simulink model "ACFT11_a_121_flatearth_backup"  (R2026a)
settings: Solver=ode15s  StopTime=10  FixedStep=0.01  MaxStep=0.05  MinStep=1e-4  AbsTol=1e-4
model workspace (MAT data in the model file):
  op11 : opcond.OperatingPoint (value not decoded)
  op_trim1 : opcond.OperatingReport (value not decoded)
  op_trim12 : opcond.OperatingReport (value not decoded)
  op_trim15 : opcond.OperatingReport (value not decoded)
  op_trim16 : opcond.OperatingReport (value not decoded)
  op_trim17 : opcond.OperatingReport (value not decoded)
  op_trim18 : opcond.OperatingReport (value not decoded)
  op_trim2 : opcond.OperatingReport (value not decoded)
  op_trim20 : opcond.OperatingReport (value not decoded)
  op_trim21 : opcond.OperatingReport (value not decoded)
  op_trim22 : opcond.OperatingReport (value not decoded)
  op_trim23 : opcond.OperatingReport (value not decoded)
  op_trim24 : opcond.OperatingReport (value not decoded)
  op_trim25 : opcond.OperatingReport (value not decoded)
  op_trim29 : opcond.OperatingReport (value not decoded)
  op_trim3 : opcond.OperatingReport (value not decoded)
  op_trim30 : opcond.OperatingReport (value not decoded)
  op_trim4 : opcond.OperatingReport (value not decoded)
  op_trim40 : opcond.OperatingReport (value not decoded)
  op_trim42 : opcond.OperatingReport (value not decoded)
  op_trim5 : opcond.OperatingReport (value not decoded)
  op_trim50 : opcond.OperatingReport (value not decoded)
  op_trim7 : opcond.OperatingReport (value not decoded)
  op_trim9 : opcond.OperatingReport (value not decoded)
values from neighbouring files (symbols this model uses):
  b = min(1, 2*(1-frac))    [export_kml.m]    (also in flight_hud.m = chaseBack; inertiatensor62.m = 9.05; setup_bfl_analysis.m = 9.05; setup_fcs_sim.m = 9.05)
  c = bar_colors{min(k,numel(bar_colors))}    [analyze_bfl.m]    (also in ecef_eom_fcn.m = w_eb_b(3); inertiatensor62.m = 15.55; optimize_indi_gains.m = 15.55; restore_normal_fcs.m = 15.55)
  CL_AlphaDot = 0    [inertiatensor62.m]    (also in setup_bfl_analysis.m; setup_fcs_sim.m; setup_takeoff_fcs.m)
  Cm_AlphaDot = 0    [inertiatensor62.m]    (also in setup_bfl_analysis.m; setup_fcs_sim.m; setup_takeoff_fcs.m)
  F = convhull(pts)    [Visualization_Takeoff2.m]    (also in attitude_ribbon.m = {[1 2 3],[1 4 2],[1 4 3],[4 5 1]})
  FCS_aerospike_thrust = 250000.0    (= 250000)    [fcs_params.m]
  FCS_alpha_max = 16.0    (= 16)    [fcs_params.m]
  FCS_bank_max = 35.0    (= 35)    [fcs_params.m]
  FCS_da_max = 20.0    (= 20)    [fcs_params.m]
  FCS_de_max = 25.0    (= 25)    [fcs_params.m]
  FCS_dr_max = 25.0    (= 25)    [fcs_params.m]
  FCS_dt = 0.01    [fcs_params.m]
  FCS_g = 9.80665    [fcs_params.m]
  FCS_Gmin_p = 0.02    [fcs_params.m]
  FCS_Gmin_q = 0.02    [fcs_params.m]
  FCS_Gmin_r = 0.01    [fcs_params.m]
  FCS_h_gnd = 2.24    [fcs_params.m]
  FCS_hdot_max = 30.0    (= 30)    [fcs_params.m]
  FCS_hdot_td = 0.3    [fcs_params.m]
  FCS_Kalpha = 3.0    (= 3)    [fcs_params.m]
  FCS_Kalpha_lim = 2.0    (= 2)    [fcs_params.m]
  FCS_Kbeta = 2.0    (= 2)    [fcs_params.m]
  FCS_Kflare = 1.0    (= 1)    [fcs_params.m]
  FCS_Kgamma = 1.5    [fcs_params.m]
  FCS_Kh = 0.10    (= 0.1)    [fcs_params.m]
  FCS_Knz = 20.0    (= 20)    [fcs_params.m]
  FCS_Kp = 6.0    (= 6)    [fcs_params.m]
  FCS_Kphi = 3.0    (= 3)    [fcs_params.m]
  FCS_Kq = 5.0    (= 5)    [fcs_params.m]
  FCS_Kr = 4.0    (= 4)    [fcs_params.m]
  FCS_Ktheta = 2.0    (= 2)    [fcs_params.m]
  FCS_link_timeout = 1.0    (= 1)    [fcs_params.m]
  FCS_MODE_AUTO = 0    [fcs_params.m]
  FCS_Nfilt = 20.0    (= 20)    [fcs_params.m]
  FCS_Nz_max = 3.0    (= 3)    [fcs_params.m]
  FCS_Nz_min = -1.0    (= -1)    [fcs_params.m]
  FCS_p_max = 40.0    (= 40)    [fcs_params.m]
  FCS_q_max = 15.0    (= 15)    [fcs_params.m]
  FCS_qbar_hi = 6000.0    (= 6000)    [fcs_params.m]
  FCS_qbar_lo = 1000.0    (= 1000)    [fcs_params.m]
  FCS_r_max = 15.0    (= 15)    [fcs_params.m]
  FCS_relight_M_hi = 2.0    (= 2)    [fcs_params.m]
  FCS_relight_M_lo = 0.35    [fcs_params.m]
  FCS_relight_qbar = 3000.0    (= 3000)    [fcs_params.m]
  FCS_stick_detent = 0.03    [fcs_params.m]
  FCS_stick_p_scale = 60.0    (= 60)    [fcs_params.m]
  FCS_stick_q_scale = 15.0    (= 15)    [fcs_params.m]
  FCS_tau_flare = 3.0    (= 3)    [fcs_params.m]
  FCS_TECS_Kep = 0.25    [fcs_params.m]
  FCS_TECS_Ktp = 0.30    (= 0.3)    [fcs_params.m]
  FCS_theta_climb = 12.0    (= 12)    [fcs_params.m]
  FCS_theta_max = 30.0    (= 30)    [fcs_params.m]
  FCS_theta_min = -20.0    (= -20)    [fcs_params.m]
  FCS_theta_trim = 0.0    (= 0)    [fcs_params.m]
  FCS_thr_max = 1.0    (= 1)    [fcs_params.m]
  FCS_thr_min = 0.0    (= 0)    [fcs_params.m]
  FCS_thr_trim = 0.50    (= 0.5)    [fcs_params.m]
  FCS_V_rotate = 94.0    (= 94)    [fcs_params.m]
  FCS_Vmin = 60.0    (= 60)    [fcs_params.m]
  FF_rates = [0.0,              2.5,              5.0,             73.0,             78.0,              0.5]    [fcs_params.m]
  g = @(n,d) i_basevar(n,d)    [analyze_control_authority.m]    (also in export_kml.m = 1 - abs(2*frac-1); inertiatensor62.m = 9.80665; setup_bfl_analysis.m = 9.80665; setup_fcs_sim.m = 9.80665)
  GS_Gp_tab = Cl_da * (S*b/Ixx)    [setup_gschedule.m]
  GS_Gq_tab = Cm_de * (S*c/Iyy)    [setup_gschedule.m]
  GS_Gr_tab = Cn_dr * (S*b/Izz)    [setup_gschedule.m]
  MASS_fuel_total = MASS_full - MASS_empty - MASS_orbiter    (= 14700)    [fcs_params.m]
  q = q/norm(q)    [build_ecef_x0.m]    (also in ecef_eom_fcn.m = state(7:10); ecef_out_fcn.m = state(7:10); setup_ecef.m; test_ecef_eom.m = state(7:10))
  r = [0;diff(xc)]/0.1    [analyze_control_authority.m]    (also in ecef_eom_fcn.m = sqrt(r_e(1)^2+r_e(2)^2+r_e(3)^2); ecef_weight_body.m = sqrt(x^2 + y^2 + z^2); export_kml.m = min(1, 2*frac); test_ecef_eom.m = sqrt(r_e(1)^2+r_e(2)^2+r_e(3)^2))
  S = {'\delta_e',DE,lim.de,'b'; '\delta_a',DA,lim.da,[0 .6 0]; '\delta_r',DR,lim.dr,[.85 .3 .1]}    [analyze_control_authority.m]    (also in attitude_ribbon.m = load(char(src)); build_ecef_x0.m = sqrt(1+C(3,3)-C(1,1)-C(2,2))*2; export_kml.m = load(char(src)); flight_hud.m = load(char(src)))
  s = A.surfaces(i)    [analyze_control_authority.m]    (also in setup_propulsion.m = [s, sprintf(')
  y_cg = 0    [inertiatensor62.m]    (also in setup_bfl_analysis.m; setup_fcs_sim.m; setup_takeoff_fcs.m)
  z_cg = 0.0    (= 0)    [inertiatensor62.m]    (also in setup_bfl_analysis.m; setup_fcs_sim.m; setup_takeoff_fcs.m)
undefined symbols (not defined in the file or in its folder): deg, DiscIntNeverNeededParam, EqM, GS_alpha_cl, GS_alpha_cm, GS_alpha_cn, GS_mach_cl, GS_mach_cm, GS_mach_cn, MIL, Moderate, rad
libraries: aerolibconvert2 x21, simulink x7, aerolibfltsims x3, aerolibwind2 x3, aerolibanim x1, aerolibatmos2 x1, shareddyn x1, aerolibobsolete x1
(part 2 of 4)

== system ACFT11_a_121_flatearth_backup/WindModels ==
  h : Inport
  V : Inport  Port=2
  DCM : Inport  Port=3
  qbar : Inport  Port=4
  phase : Inport  Port=5
  DiscreteGust : aerolibwind2/Discrete Wind Gust Model  units=Metric (MKS)  Gx=on  Gy=on  Gz=on  t_0=WIND_gust_t0  d_m=WIND_gust_len  v_m=WIND_gust_amp
  Dryden Wind Turbulence Model (Discrete (+q +r)) : aerolibwind2/Dryden Wind Turbulence Model  (Continuous (+q -r))  units=Metric (MKS)  spec=MIL-F-8785C  model=Discrete Dryden (+q +r)  W20=WIND_W20  Wdeg=WIND_Wdeg  TurbProb=10^-3 - Moderate  L_high=WIND_Lhigh  Wingspan=FCS_b  ts=0.02  Seed=[23341 23342 23343 23344]  T_on=on
      settings: LibrarySourceBlock=|
      | aerolibwind2/Dryden Wind Turbulence Model
      | (Discrete (+q +r))
  MeanToBody : Product  Multiplication=Matrix(*)
  MeanWind : MATLAB Function  TreatAsAtomicUnit=on
  Scheduler : MATLAB Function  TreatAsAtomicUnit=on
  Vclamp : Saturate  UpperLimit=inf  LowerLimit=1
  WindShear : aerolibwind2/Wind Shear Model  units=Metric (MKS)  phase=Category C - Terminal Flight Phase  W_20=WIND_W20  Wdeg=WIND_Wdeg
  gDemux : Demux  Outputs=3
  pGust : Product
  pRate : Product
  pShear : Product
  pTurb : Product
  sWind : Sum  Inputs=++++
  WindBody : Outport
  GustRates : Outport  Port=2
  wires:
  V/1 -> Vclamp/1
  h/1 -> Dryden Wind Turbulence Model (Discrete (+q +r))/1, WindShear/1, MeanWind/1(h), Scheduler/3(h)
  Vclamp/1 -> Dryden Wind Turbulence Model (Discrete (+q +r))/2, DiscreteGust/1
  DCM/1 -> Dryden Wind Turbulence Model (Discrete (+q +r))/3, WindShear/2, MeanToBody/1
  MeanWind/1(W_ned) -> MeanToBody/2
  qbar/1 -> Scheduler/1(qbar)
  phase/1 -> Scheduler/2(phase)
  Scheduler/1(g) -> gDemux/1
  gDemux/1 -> pTurb/2, pRate/2
  gDemux/2 -> pGust/2
  gDemux/3 -> pShear/2
  Dryden Wind Turbulence Model (Discrete (+q +r))/1 -> pTurb/1
  Dryden Wind Turbulence Model (Discrete (+q +r))/2 -> pRate/1
  WindShear/1 -> pShear/1
  DiscreteGust/1 -> pGust/1
  MeanToBody/1 -> sWind/1
  pTurb/1 -> sWind/2
  pShear/1 -> sWind/3
  pGust/1 -> sWind/4
  sWind/1 -> WindBody/1
  pRate/1 -> GustRates/1

== system ACFT11_a_121_flatearth_backup/aerospike ==
  Manual Switch1 : ManualSwitch
  Scope1 : Scope
      settings: ActiveDisplayYMinimum=711.4  ActiveDisplayYMaximum=2711.4  DataLoggingVariableName=ScopeData8
  TotalWeight full : Constant  Value=24000
  TotalWeightempty : Constant  Value=10800
  net mass : Outport
  wires:
  TotalWeight full/1 -> Manual Switch1/1
  Manual Switch1/1 -> net mass/1, Scope1/1
  TotalWeightempty/1 -> Manual Switch1/2

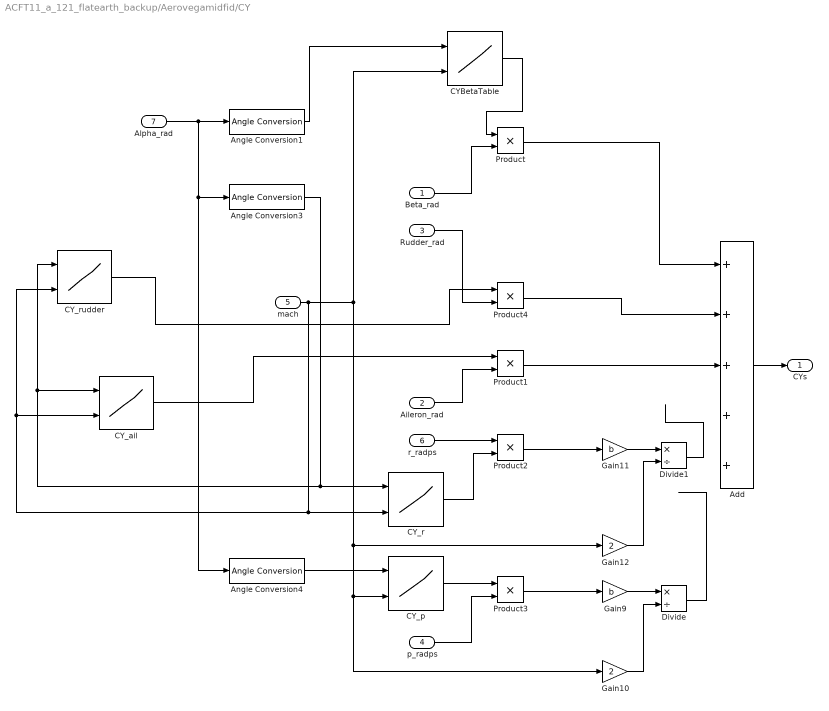
== system ACFT11_a_121_flatearth_backup/Aerovegamidfid/CY ==
  Beta_rad : Inport
  Aileron_rad : Inport  Port=2
  Rudder_rad : Inport  Port=3
  p_radps : Inport  Port=4
  mach : Inport  Port=5
  r_radps : Inport  Port=6
  Alpha_rad : Inport  Port=7
  Add : Sum  Inputs=+++++
  Angle Conversion1 : aerolibconvert2/Angle Conversion  IU=rad  OU=deg
  Angle Conversion3 : aerolibconvert2/Angle Conversion  IU=rad  OU=deg
  Angle Conversion4 : aerolibconvert2/Angle Conversion  IU=rad  OU=deg
  CYBetaTable : Lookup_n-D  BreakpointsForDimension1=[-10;-5;0;5;10;15;20]  BreakpointsForDimension2=[0.40000000000000002;0.59999999999999998;0.80000000000000004;0.90000000000000002;0.94999999999999996;1;1.05;1.1000000000000001;1.1499999999999999;1.2;1.3999999999999999;1.6000000000000001;1.8;2;2.2000000000000002;2.3999999999999999;2.6000000000000001;2.7999999999999998;3;3.2000000000000002;3.3999999999999999;3.6000000000000001;3.7999999999999998;4]  Table=[-0.12776999999999999 -0.15103 -0.19447999999999999 -0.19447999999999999 -0.19447999999999999 -0.23501 -0.24235000000000001 -0.24121000000000001 -0.23999000000000001 -0.23599999999999999 -0.23136000000000001 -0.22819 -0.22448000000000001 -0.22019 -0.22012000000000001 -0.22012000000000001 -0.22312000000000001 -0.22312000000000001 -0.21296999999999999 -0.20682 -0.20682 -0.20682 -0.20682 -0.20682;-0.13353000000000001 -0.13844999999999999 -0.1512 -0.17480999999999999 -0.20491000000000001 -0.23100999999999999 -0.22816 -0.21564 -0.20358999999999999 -0.19808999999999999 -0.22040000000000001 -0.20463000000000001 -0.19264000000000001 -0.19131999999999999 -0.19667000000000001 -0.19667000000000001 -0.1976 -0.1976 -0.19153000000000001 -0.18745999999999999 -0.18447 -0.18074999999999999 -0.17644000000000001 -0.17335;-0.12477000000000001 -0.12477000000000001 -0.14726 -0.18393000000000001 -0.19086 -0.25681999999999999 -0.2135 -0.20412 -0.19841 -0.18865000000000001 -0.18257000000000001 -0.18975 -0.18453 -0.17534 -0.16897999999999999 -0.16897999999999999 -0.16542000000000001 -0.16542000000000001 -0.16613 -0.1658 -0.16546 -0.16469 -0.16469 -0.16008;-0.14713999999999999 -0.15239 -0.16939000000000001 -0.17382 -0.16824 -0.26501999999999998 -0.23901 -0.23458000000000001 -0.21525 -0.20416000000000001 -0.19020000000000001 -0.19077 -0.19361999999999999 -0.19001999999999999 -0.18447 -0.18447 -0.18201999999999999 -0.18201999999999999 -0.18214 -0.18174000000000001 -0.18174000000000001 -0.17979000000000001 -0.17979000000000001 -0.17630999999999999;0.027699999999999999 -0.03637 -0.15801000000000001 -0.15759999999999999 -0.16692000000000001 -0.17283000000000001 -0.18171000000000001 -0.17918999999999999 -0.18587999999999999 -0.19109000000000001 -0.19761000000000001 -0.19316 -0.21625 -0.20916000000000001 -0.21368000000000001 -0.21368000000000001 -0.21557999999999999 -0.21557999999999999 -0.21690000000000001 -0.21461 -0.21259 -0.21259 -0.21259 -0.21259;-0.11840000000000001 -0.11840000000000001 -0.10925 -0.17466999999999999 -0.14785000000000001 -0.22763 -0.22448000000000001 -0.21309 -0.20909 -0.20437 -0.21088999999999999 -0.20282 -0.20863000000000001 -0.21868000000000001 -0.22735 -0.22735 -0.23788999999999999 -0.23788999999999999 -0.24143999999999999 -0.23699000000000001 -0.23699000000000001 -0.23308000000000001 -0.2301 -0.22547;0.109066 0.109066 0.053113 -0.11154 -0.1827 -0.16996 -0.17655000000000001 -0.18178 -0.18887999999999999 -0.18886 -0.20727999999999999 -0.22977 -0.23341000000000001 -0.23487 -0.23748 -0.23748 -0.24157999999999999 -0.24157999999999999 -0.24506 -0.24368000000000001 -0.24368000000000001 -0.24495 -0.24395 -0.24395]  InternalRulePriority=Speed  RndMeth=Simplest
      settings: InputPortMap=u0,u1
  CY_ail : Lookup_n-D  BreakpointsForDimension1=[-10;-5;0;5;10;15;20]  BreakpointsForDimension2=[0.40000000000000002;0.59999999999999998;0.80000000000000004;0.90000000000000002;0.94999999999999996;1;1.05;1.1000000000000001;1.1499999999999999;1.2;1.3999999999999999;1.6000000000000001;1.8;2;2.2000000000000002;2.3999999999999999;2.6000000000000001;2.7999999999999998;3;3.2000000000000002]  Table=[-0.043959999999999999 -0.049730000000000003 -0.089330000000000007 -0.049299999999999997 -0.060999999999999999 -0.0050099999999999997 -0.0059800000000000001 -0.0063699999999999998 -0.0053200000000000001 -0.0047200000000000002 -2.0999999999999999e-05 0.005326 0.0074289999999999998 0.0077289999999999998 0.0074089999999999998 0.0074089999999999998 0.0066439999999999997 0.0066439999999999997 0.0057539999999999996 0.0044730000000000004;-0.045089999999999998 -0.04623 -0.07195 -0.090139999999999998 -0.066970000000000002 -0.0040800000000000003 -0.00172 -0.0018699999999999999 -0.00036999999999999999 0.0027390000000000001 0.0094590000000000004 0.010628 0.0099010000000000001 0.0089040000000000005 0.0080180000000000008 0.0072870000000000001 0.0066829999999999997 0.0060340000000000003 0.0054229999999999999 0.004816;-0.024709999999999999 -0.028559999999999999 -0.029700000000000001 -0.022249999999999999 -0.067199999999999996 0.001359 0.0094889999999999992 0.01074 0.011264 0.011575 0.011604 0.011159000000000001 0.0097300000000000008 0.0060169999999999998 0.0074250000000000002 0.0066429999999999996 0.0060029999999999997 0.0054050000000000001 0.0049160000000000002 0.0043969999999999999;-0.0086800000000000002 -0.0079100000000000004 0.0050159999999999996 -0.058790000000000002 0.043109000000000001 0.014027 0.0088889999999999993 0.011901 0.013266999999999999 0.013504 0.011289 0.01005 0.0091170000000000001 0.0078560000000000001 0.0069020000000000001 0.0061529999999999996 0.0055189999999999996 0.0049569999999999996 0.0045659999999999997 0.0041679999999999998;0.041435 0.014364 -0.0019400000000000001 -0.00464 -0.01489 -0.01 -0.017180000000000001 -0.013010000000000001 -0.0077600000000000004 -0.0022300000000000002 0.00413 0.0053379999999999999 0.0054580000000000002 0.0056649999999999999 0.0058910000000000004 0.0055620000000000001 0.0051310000000000001 0.0045799999999999999 0.0044580000000000002 0.0045950000000000001;0.030383 -0.0082000000000000007 -0.00066 -0.019890000000000001 -0.02223 -0.01924 -0.01474 -0.012109999999999999 -0.01082 -0.0053499999999999997 0.0059630000000000004 0.0064679999999999998 0.0061799999999999997 0.005633 0.0059040000000000004 0.0062199999999999998 0.006352 0.0058929999999999998 0.0058809999999999999 0.0055579999999999996;0.035274 0.035754000000000001 0.10789799999999999 0.107908 -0.018100000000000002 -0.01762 -0.01268 -0.0087100000000000007 -0.0064400000000000004 -0.00379 0.0063749999999999996 0.0080339999999999995 0.007587 0.0075339999999999999 0.00762 0.0074390000000000003 0.0074419999999999998 0.0071830000000000001 0.0069100000000000003 0.0081550000000000008]  InternalRulePriority=Speed  RndMeth=Simplest
      settings: InputPortMap=u0,u1
  CY_p : Lookup_n-D  BreakpointsForDimension1=[-4;4;12;20]  BreakpointsForDimension2=[134;809]  Table=[-0.1770962 -0.0487863;0.11228 0.0438075;0.4040726 0.135549;0.6897346 0.2246525]  InternalRulePriority=Speed  RndMeth=Simplest
      settings: InputPortMap=u0,u1
  CY_r : Lookup_n-D  BreakpointsForDimension1=[-4;4;12;20]  BreakpointsForDimension2=[134;809]  Table=[0.1493543 0.1366935;0.1608132 0.1063935;0.1691043 0.0740228;0.1777061 0.0402114]  InternalRulePriority=Speed  RndMeth=Simplest
      settings: InputPortMap=u0,u1
  CY_rudder : Lookup_n-D  BreakpointsForDimension1=[-5;0;5;10;15;20]  BreakpointsForDimension2=[0.40000000000000002;0.59999999999999998;0.80000000000000004;0.90000000000000002;0.94999999999999996;1;1.05;1.1000000000000001;1.1499999999999999;1.2;1.3999999999999999;1.6000000000000001;1.8;2;2.2000000000000002;2.3999999999999999;2.6000000000000001;2.7999999999999998;3;3.2000000000000002;3.3999999999999999;3.6000000000000001;3.7999999999999998;4]  Table=[0.076880000000000004 0.078581999999999999 0.077237 0.077237 0.077237 0.069614999999999996 0.064549999999999996 0.060617999999999998 0.056524999999999999 0.052881999999999998 0.041794999999999999 0.034744999999999998 0.030259000000000001 0.027265000000000001 0.024920999999999999 0.022969 0.021485000000000001 0.020365000000000001 0.019557000000000001 0.019557000000000001 0.017876 0.017388000000000001 0.017066000000000001 0.016771000000000001;0.071577000000000002 0.072626999999999997 0.073166999999999996 0.064906000000000005 0.064906000000000005 0.062094000000000003 0.063351000000000005 0.060872999999999997 0.057183999999999999 0.053927999999999997 0.041528000000000002 0.033975999999999999 0.028912 0.024951999999999998 0.022040000000000001 0.019795 0.017974 0.016538000000000001 0.015436999999999999 0.015436999999999999 0.013459 0.012857 0.0124 0.012049000000000001;0.075864000000000001 0.079436000000000007 0.077657000000000004 0.077657000000000004 0.077657000000000004 0.053987 0.043984000000000002 0.041881000000000002 0.041881000000000002 0.051196999999999999 0.039151999999999999 0.031641000000000002 0.025566999999999999 0.021420000000000002 0.018223 0.015931000000000001 0.014336 0.013115999999999999 0.012099 0.012099 0.010333 0.009776 0.009358 0.0089759999999999996;0.061571000000000001 0.074791999999999997 0.063759999999999997 0.065167000000000003 0.065167000000000003 0.065167000000000003 0.053246000000000002 0.051076000000000003 0.047258000000000001 0.043964999999999997 0.033118000000000002 0.025888999999999999 0.01942 0.015737000000000001 0.013604 0.012597000000000001 0.011712 0.010699 0.0099240000000000005 0.0099240000000000005 0.008567 0.0079839999999999998 0.0076290000000000004 0.007365;0.046331999999999998 0.053748999999999998 0.061512999999999998 0.055087999999999998 0.055087999999999998 0.059921000000000002 0.055232999999999997 0.051126999999999999 0.046517000000000003 0.041138000000000001 0.030085000000000001 0.023015999999999998 0.018096000000000001 0.014723 0.012234999999999999 0.010198 0.010198 0.010198 0.0083129999999999992 0.0083129999999999992 0.0071710000000000003 0.0068599999999999998 0.0066 0.006326;0.043413 0.043413 0.061019999999999998 0.055966000000000002 0.076019000000000003 0.063729999999999995 0.056828999999999998 0.052475000000000001 0.047745000000000003 0.041173000000000001 0.027605000000000001 0.020657999999999999 0.015854 0.012926 0.010586999999999999 0.0091660000000000005 0.0077710000000000001 0.0077710000000000001 0.0077710000000000001 0.0077710000000000001 0.0058060000000000004 0.0057000000000000002 0.0055050000000000003 0.0055050000000000003]  InternalRulePriority=Speed  RndMeth=Simplest
      settings: InputPortMap=u0,u1
  Divide : Product  Inputs=*/
  Divide1 : Product  Inputs=*/
  Gain10 : Gain  Gain=2
  Gain11 : Gain  Gain=b
  Gain12 : Gain  Gain=2
  Gain9 : Gain  Gain=b
  Product{,1..4} (5 alike) : Product
  CYs : Outport
  wires:
  Beta_rad/1 -> Product/2
  mach/1 -> CY_r/2, CY_rudder/2, CY_ail/2, CYBetaTable/2, Gain10/1, CY_p/2, Gain12/1
  Rudder_rad/1 -> Product4/2
  Angle Conversion3/1 -> CY_r/1, CY_rudder/1, CY_ail/1
  Alpha_rad/1 -> Angle Conversion3/1, Angle Conversion4/1, Angle Conversion1/1
  CYBetaTable/1 -> Product/1
  Angle Conversion1/1 -> CYBetaTable/1
  Angle Conversion4/1 -> CY_p/1
  CY_rudder/1 -> Product4/1
  CY_ail/1 -> Product1/1
  Aileron_rad/1 -> Product1/2
  r_radps/1 -> Product2/1
  CY_r/1 -> Product2/2
  CY_p/1 -> Product3/1
  p_radps/1 -> Product3/2
  Product/1 -> Add/1
  Divide1/1 -> ?
  Product4/1 -> Add/2
  Product1/1 -> Add/3
  Product2/1 -> Gain11/1
  Divide/1 -> ?
  Product3/1 -> Gain9/1
  Gain11/1 -> Divide1/1
  Gain12/1 -> Divide1/2
  Gain9/1 -> Divide/1
  Gain10/1 -> Divide/2
  Add/1 -> CYs/1

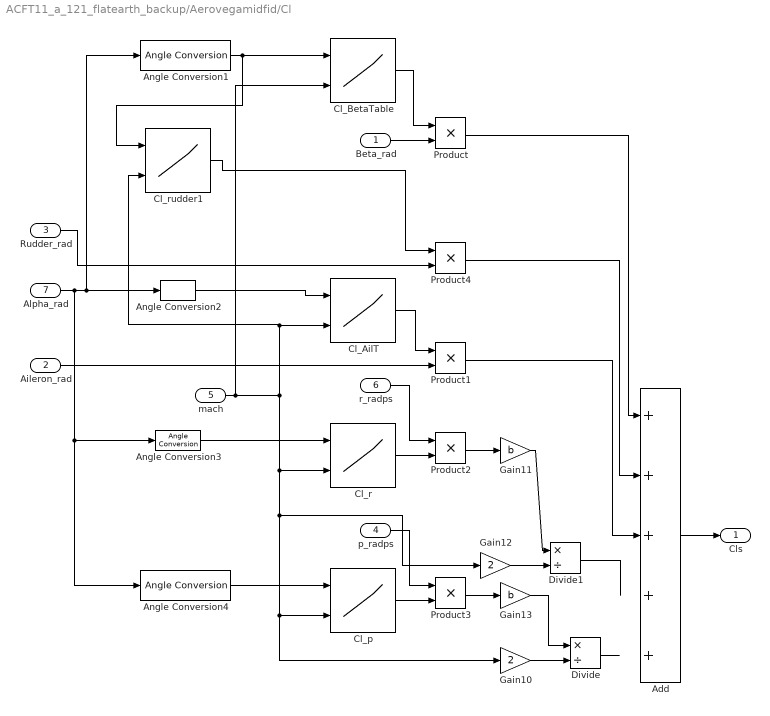
== system ACFT11_a_121_flatearth_backup/Aerovegamidfid/Cl ==
  Beta_rad : Inport
  Aileron_rad : Inport  Port=2
  Rudder_rad : Inport  Port=3
  p_radps : Inport  Port=4
  mach : Inport  Port=5
  r_radps : Inport  Port=6
  Alpha_rad : Inport  Port=7
  Add : Sum  Inputs=+++++
  Angle Conversion{1..4} (4 alike) : aerolibconvert2/Angle Conversion  IU=rad  OU=deg
  Cl_AilT : Lookup_n-D  BreakpointsForDimension1=[-10;-5;0;5;10;15;20]  BreakpointsForDimension2=[0.40000000000000002;0.59999999999999998;0.80000000000000004;0.90000000000000002;0.94999999999999996;1;1.05;1.1000000000000001;1.1499999999999999;1.2;1.3999999999999999;1.6000000000000001;1.8;2;2.2000000000000002;2.3999999999999999;2.6000000000000001;2.7999999999999998;3;3.2000000000000002]  BreakpointsForDimension3=[10 20 30]  Table=[-0.12067 -0.13686999999999999 -0.16031000000000001 -0.12655 -0.13017000000000001 -0.088929999999999995 -0.084239999999999995 -0.079479999999999995 -0.073959999999999998 -0.069370000000000001 -0.05178 -0.040079999999999998 -0.033050000000000003 -0.02809 -0.02445 -0.02445 -0.01975 -0.01975 -0.016299999999999999 -0.01448;-0.11831999999999999 -0.12526000000000001 -0.14226 -0.16092000000000001 -0.14421 -0.091240000000000002 -0.087609999999999993 -0.082110000000000002 -0.075090000000000004 -0.068510000000000001 -0.052720000000000003 -0.041930000000000002 -0.0344 -0.0292 -0.025340000000000001 -0.0224 -0.019800000000000002 -0.017479999999999999 -0.015520000000000001 -0.013650000000000001;-0.12389 -0.13103000000000001 -0.13703000000000001 -0.12989000000000001 -0.13633999999999999 -0.073419999999999999 -0.082869999999999999 -0.076630000000000004 -0.069500000000000006 -0.063060000000000005 -0.048329999999999998 -0.039320000000000001 -0.032140000000000002 -0.0269 -0.023109999999999999 -0.02026 -0.01797 -0.0161 -0.01447 -0.01282;-0.12914 -0.12986 -0.12119000000000001 -0.12909000000000001 -0.10125000000000001 -0.067059999999999995 -0.084000000000000005 -0.077210000000000001 -0.069029999999999994 -0.061879999999999998 -0.044819999999999999 -0.036150000000000002 -0.029860000000000001 -0.024979999999999999 -0.021430000000000001 -0.018710000000000001 -0.016629999999999999 -0.01494 -0.01358 -0.012200000000000001;-0.096979999999999997 -0.1246 -0.13456000000000001 -0.11885999999999999 -0.10561 -0.081909999999999997 -0.08165 -0.077009999999999995 -0.06923 -0.062509999999999996 -0.040669999999999998 -0.03117 -0.02596 -0.022329999999999999 -0.019400000000000001 -0.01728 -0.01566 -0.01457 -0.013729999999999999 -0.01315;-0.094140000000000001 -0.14399000000000001 -0.13264999999999999 -0.13927 -0.10493 -0.084449999999999997 -0.078049999999999994 -0.071749999999999994 -0.065850000000000006 -0.05987 -0.040169999999999997 -0.028889999999999999 -0.024590000000000001 -0.02256 -0.020889999999999999 -0.019480000000000001 -0.017919999999999998 -0.016920000000000001 -0.016119999999999999 -0.01529;-0.11415 -0.10864 -0.14979999999999999 -0.15307000000000001 -0.085010000000000002 -0.081439999999999999 -0.073760000000000006 -0.070510000000000003 -0.066659999999999997 -0.061289999999999997 -0.045269999999999998 -0.034079999999999999 -0.027279999999999999 -0.024420000000000001 -0.02307 -0.02247 -0.021520000000000001 -0.02086 -0.020150000000000001 -0.020590000000000001]  InternalRulePriority=Speed  RndMeth=Simplest
      settings: InputPortMap=u0,u1
  Cl_BetaTable : Lookup_n-D  BreakpointsForDimension1=[-10;-5;0;5;10;15;20]  BreakpointsForDimension2=[0.40000000000000002;0.59999999999999998;0.80000000000000004;0.90000000000000002;0.94999999999999996;1;1.05;1.1000000000000001;1.1499999999999999;1.2;1.3999999999999999;1.6000000000000001;1.8;2;2.2000000000000002;2.3999999999999999;2.6000000000000001;2.7999999999999998;3;3.2000000000000002;3.3999999999999999;3.6000000000000001;3.7999999999999998;4]  Table=[0.092985999999999999 0.073393 0.095170000000000005 0.095170000000000005 0.095170000000000005 0.084915000000000004 0.088636000000000006 0.083512000000000003 0.079314999999999997 0.074557999999999999 0.066761000000000001 0.062025999999999998 0.063884999999999997 0.064086000000000004 0.059843 0.059843 0.047805 0.047805 0.03952 0.037555999999999999 0.037555999999999999 0.037555999999999999 0.037555999999999999 0.037555999999999999;0.051325999999999997 0.049796 0.040059999999999998 0.028015999999999999 0.031426999999999997 0.037841 0.035071999999999999 0.03628 0.037296999999999997 0.035583999999999998 0.030606000000000001 0.022492999999999999 0.019574000000000001 0.023470999999999999 0.027022000000000001 0.027022000000000001 0.026016000000000001 0.026016000000000001 0.021356 0.019550999999999999 0.019480999999999998 0.019230000000000001 0.019064999999999999 0.019453000000000002;-0.029530000000000001 -0.029530000000000001 -0.041279999999999997 -0.049660000000000003 -0.040070000000000001 -0.02852 -0.026290000000000001 -0.029680000000000002 -0.031140000000000001 -0.029700000000000001 -0.02895 -0.02963 -0.03243 -0.029579999999999999 -0.024410000000000001 -0.024410000000000001 -0.0109 -0.0109 -0.00181 -5.7000000000000003e-05 0.001333 0.0025720000000000001 0.0025720000000000001 0.0038600000000000001;-0.11409 -0.11309 -0.12584000000000001 -0.12203 -0.10780000000000001 -0.1166 -0.089940000000000006 -0.092649999999999996 -0.093850000000000003 -0.096680000000000002 -0.096869999999999998 -0.086870000000000003 -0.077840000000000006 -0.069080000000000003 -0.059150000000000001 -0.059150000000000001 -0.041300000000000003 -0.041300000000000003 -0.027459999999999998 -0.022919999999999999 -0.022919999999999999 -0.017510000000000001 -0.017510000000000001 -0.015389999999999999;-0.068290000000000003 -0.11047 -0.18926000000000001 -0.18806999999999999 -0.15681999999999999 -0.14993999999999999 -0.14585000000000001 -0.13827999999999999 -0.13611000000000001 -0.13924 -0.14846999999999999 -0.14316999999999999 -0.12834000000000001 -0.099400000000000002 -0.087870000000000004 -0.087870000000000004 -0.066439999999999999 -0.066439999999999999 -0.054300000000000001 -0.05049 -0.046429999999999999 -0.046429999999999999 -0.046429999999999999 -0.046429999999999999;-0.30023 -0.30023 -0.28955999999999998 -0.29981000000000002 -0.23200999999999999 -0.23960000000000001 -0.22 -0.20660999999999999 -0.19647000000000001 -0.18243000000000001 -0.16672000000000001 -0.15804000000000001 -0.14368 -0.12787000000000001 -0.10843 -0.10843 -0.087300000000000003 -0.087300000000000003 -0.078570000000000001 -0.076399999999999996 -0.076399999999999996 -0.069349999999999995 -0.066379999999999995 -0.064079999999999998;-0.30027999999999999 -0.30027999999999999 -0.34923999999999999 -0.31956000000000001 -0.30431999999999998 -0.26140999999999998 -0.24820999999999999 -0.23746999999999999 -0.22319 -0.20755000000000001 -0.16458999999999999 -0.15185999999999999 -0.13661999999999999 -0.12536 -0.11414000000000001 -0.11414000000000001 -0.097420000000000007 -0.097420000000000007 -0.092050000000000007 -0.09035 -0.09035 -0.08949 -0.088260000000000005 -0.088260000000000005]  InternalRulePriority=Speed  RndMeth=Simplest
      settings: InputPortMap=u0,u1
  Cl_p : Lookup_n-D  BreakpointsForDimension1=[-4;4;12;20]  BreakpointsForDimension2=[134;809]  Table=[-0.1161233 -0.1096215;-0.1227074 -0.1216723;-0.1360891 -0.1313548;-0.1551817 -0.1384806]  InternalRulePriority=Speed  RndMeth=Simplest
      settings: InputPortMap=u0,u1
  Cl_r : Lookup_n-D  BreakpointsForDimension1=[-4;4;12;20]  BreakpointsForDimension2=[134;809]  Table=[-0.07000149999999999 -0.0729803;0.074753 0.0249366;0.2173445 0.1223684;0.3545122 0.2174183]  InternalRulePriority=Speed  RndMeth=Simplest
      settings: InputPortMap=u0,u1
  Cl_rudder1 : Lookup_n-D  BreakpointsForDimension1=[-5;0;5;10;15;20]  BreakpointsForDimension2=[0.40000000000000002;0.59999999999999998;0.80000000000000004;0.90000000000000002;0.94999999999999996;1;1.05;1.1000000000000001;1.1499999999999999;1.2;1.3999999999999999;1.6000000000000001;1.8;2;2.2000000000000002;2.3999999999999999;2.6000000000000001;2.7999999999999998;3;3.2000000000000002;3.3999999999999999;3.6000000000000001;3.7999999999999998;4]  Table=[0.025825000000000001 0.027431000000000001 0.029722999999999999 0.029722999999999999 0.029722999999999999 0.011398 0.012862999999999999 0.012042000000000001 0.011328 0.010538 0.0075900000000000004 0.0060870000000000004 0.005254 0.0047210000000000004 0.0042890000000000003 0.003947 0.0036779999999999998 0.0034849999999999998 0.0033600000000000001 0.0033600000000000001 0.0030769999999999999 0.0029979999999999998 0.002954 0.0029239999999999999;0.028006 0.028916000000000001 0.030297000000000001 0.027408999999999999 0.027408999999999999 0.013620999999999999 0.012741000000000001 0.012004000000000001 0.011609 0.010599000000000001 0.0080829999999999999 0.0063480000000000003 0.0053610000000000003 0.0045979999999999997 0.0040610000000000004 0.0036359999999999999 0.0032799999999999999 0.0030010000000000002 0.0027910000000000001 0.0027910000000000001 0.0024510000000000001 0.002323 0.0022469999999999999 0.0021789999999999999;0.031910000000000001 0.032996999999999999 0.031847 0.031847 0.031847 0.016813000000000002 0.0084600000000000005 0.0072459999999999998 0.0072459999999999998 0.009979 0.007816 0.0061539999999999997 0.0049529999999999999 0.004143 0.0035469999999999998 0.003127 0.0027850000000000001 0.002526 0.0023210000000000001 0.0023210000000000001 0.0019910000000000001 0.0019040000000000001 0.0018129999999999999 0.0017420000000000001;0.024653999999999999 0.030564000000000001 0.025260999999999999 0.024257000000000001 0.024257000000000001 0.024257000000000001 0.010978 0.010003 0.0095569999999999995 0.0087320000000000002 0.0062379999999999996 0.0048669999999999998 0.0036879999999999999 0.0031350000000000002 0.0026540000000000001 0.0024350000000000001 0.0023249999999999998 0.0021289999999999998 0.0019629999999999999 0.0019629999999999999 0.001709 0.0015900000000000001 0.0015020000000000001 0.001439;0.017936000000000001 0.022425 0.023408000000000002 0.018044000000000001 0.018044000000000001 0.011950000000000001 0.010976 0.010442999999999999 0.0091280000000000007 0.0082470000000000009 0.0058799999999999998 0.004313 0.0034020000000000001 0.0028029999999999999 0.0023999999999999998 0.001933 0.001933 0.001933 0.001621 0.001621 0.0015399999999999999 0.001426 0.0013060000000000001 0.0012110000000000001;0.018714000000000001 0.018714000000000001 0.022092000000000001 0.018027999999999999 0.020263 0.014347 0.012631 0.011469 0.010281 0.0088769999999999995 0.0055180000000000003 0.004006 0.0030460000000000001 0.0024429999999999999 0.0021419999999999998 0.0020100000000000001 0.0017830000000000001 0.0017830000000000001 0.0017830000000000001 0.0017830000000000001 0.0011640000000000001 0.0012260000000000001 0.0011119999999999999 0.0011119999999999999]  InternalRulePriority=Speed  RndMeth=Simplest
      settings: InputPortMap=u0,u1
  Divide : Product  Inputs=*/
  Divide1 : Product  Inputs=*/
  Gain10 : Gain  Gain=2
  Gain11 : Gain  Gain=b
  Gain12 : Gain  Gain=2
  Gain13 : Gain  Gain=b
  Product{,1..4} (5 alike) : Product
  Cls : Outport
  wires:
  Aileron_rad/1 -> Product1/2
  Rudder_rad/1 -> Product4/2
  Cl_BetaTable/1 -> Product/1
  mach/1 -> Gain10/1, Cl_p/2, Gain12/1, Cl_r/2, Cl_rudder1/2, Cl_AilT/2, Cl_BetaTable/2
  Gain13/1 -> Divide/1
  Angle Conversion1/1 -> Cl_rudder1/1, Cl_BetaTable/1
  Cl_p/1 -> Product3/2
  Angle Conversion3/1 -> Cl_r/1
  Alpha_rad/1 -> Angle Conversion4/1, Angle Conversion3/1, Angle Conversion2/1, Angle Conversion1/1
  Angle Conversion2/1 -> Cl_AilT/1
  Product1/1 -> Add/3
  Angle Conversion4/1 -> Cl_p/1
  Beta_rad/1 -> Product/2
  Cl_rudder1/1 -> Product4/1
  Cl_AilT/1 -> Product1/1
  r_radps/1 -> Product2/1
  Add/1 -> Cls/1
  Gain11/1 -> Divide1/1
  Cl_r/1 -> Product2/2
  p_radps/1 -> Product3/1
  Product/1 -> Add/1
  Product4/1 -> Add/2
  Product2/1 -> Gain11/1
  Product3/1 -> Gain13/1
  Divide/1 -> ?
  Gain12/1 -> Divide1/2
  Gain10/1 -> Divide/2
  Divide1/1 -> ?

== system ACFT11_a_121_flatearth_backup/Aerovegamidfid/Cm ==
  Alpha_rad : Inport
  Elevator_rad : Inport  Port=2
  AlphaDot_radps : Inport  Port=3
  q_radps : Inport  Port=4
  mach : Inport  Port=5
  Add : Sum  Inputs=++++
  Angle Conversion1 : aerolibconvert2/Angle Conversion  IU=rad  OU=deg
  Angle Conversion2 : aerolibconvert2/Angle Conversion  IU=rad  OU=deg
  Angle Conversion3 : aerolibconvert2/Angle Conversion  IU=rad  OU=deg
  Cm_elev : Lookup_n-D  BreakpointsForDimension1=[-10;-5;0;5;10;15;20]  BreakpointsForDimension2=[0;0.40000000000000002;0.59999999999999998;0.80000000000000004;0.90000000000000002;0.94999999999999996;1;1.05;1.1000000000000001;1.1499999999999999;1.2;1.3999999999999999;1.6000000000000001;1.8;2;2.2000000000000002;2.3999999999999999;2.6000000000000001;2.7999999999999998;3;3.2000000000000002;3.3999999999999999;3.6000000000000001;3.7999999999999998;4]  BreakpointsForDimension3=[10 20 30]  Table=[-0.13624 -0.13624 -0.15662000000000001 -0.18164 -0.16969000000000001 -0.17082 -0.12374 -0.11055 -0.10353999999999999 -0.095949999999999994 -0.089020000000000002 -0.066299999999999998 -0.051970000000000002 -0.043150000000000001 -0.036769999999999997 -0.032070000000000001 -0.032070000000000001 -0.025669999999999998 -0.025669999999999998 -0.021190000000000001 -0.01925 -0.01925 -0.01925 -0.01925 -0.01925;-0.13550000000000001 -0.13550000000000001 -0.14635999999999999 -0.17236000000000001 -0.20549000000000001 -0.20075999999999999 -0.11788 -0.11283 -0.10555 -0.096199999999999994 -0.087620000000000003 -0.068000000000000005 -0.054460000000000001 -0.044850000000000001 -0.038080000000000003 -0.033000000000000002 -0.029139999999999999 -0.02581 -0.022870000000000001 -0.02035 -0.01787 -0.01537 -0.013939999999999999 -0.01281 -0.01174;-0.14179 -0.14179 -0.15337000000000001 -0.17099 -0.17593 -0.18798999999999999 -0.098790000000000003 -0.10929999999999999 -0.10108 -0.091700000000000004 -0.082790000000000002 -0.062920000000000004 -0.051290000000000002 -0.042209999999999998 -0.035860000000000003 -0.030519999999999999 -0.026700000000000002 -0.023689999999999999 -0.021219999999999999 -0.019060000000000001 -0.01685 -0.014659999999999999 -0.01323 -0.01205 -0.01098;-0.14704999999999999 -0.14704999999999999 -0.15357999999999999 -0.15820999999999999 -0.17527000000000001 -0.14652999999999999 -0.092079999999999995 -0.1111 -0.10256999999999999 -0.091939999999999994 -0.082049999999999998 -0.05917 -0.047690000000000003 -0.039440000000000003 -0.033180000000000001 -0.028549999999999999 -0.024979999999999999 -0.022179999999999998 -0.019859999999999999 -0.017950000000000001 -0.0161 -0.01434 -0.01319 -0.0123 -0.011520000000000001;-0.11999 -0.11999 -0.14879000000000001 -0.17377000000000001 -0.16980999999999999 -0.14943999999999999 -0.11021 -0.10624 -0.10063999999999999 -0.09085 -0.082729999999999998 -0.054469999999999998 -0.041770000000000002 -0.034590000000000003 -0.029649999999999999 -0.025819999999999999 -0.02308 -0.020809999999999999 -0.019220000000000001 -0.018010000000000002 -0.01754 -0.015720000000000001 -0.01507 -0.014420000000000001 -0.01388;-0.11446000000000001 -0.11446000000000001 -0.16705 -0.17222999999999999 -0.19719999999999999 -0.14104 -0.11197 -0.10390000000000001 -0.095430000000000001 -0.087139999999999995 -0.079130000000000006 -0.05355 -0.038429999999999999 -0.032419999999999997 -0.02886 -0.027349999999999999 -0.025760000000000002 -0.023800000000000002 -0.02248 -0.021489999999999999 -0.020299999999999999 -0.019599999999999999 -0.019109999999999999 -0.01866 -0.018239999999999999;-0.12103999999999999 -0.12103999999999999 -0.13317000000000001 -0.15365000000000001 -0.18323 -0.11380999999999999 -0.10419 -0.096329999999999999 -0.092490000000000003 -0.088499999999999995 -0.081509999999999999 -0.059639999999999999 -0.044999999999999998 -0.03576 -0.032160000000000001 -0.030380000000000001 -0.029559999999999999 -0.028379999999999999 -0.027490000000000001 -0.026530000000000001 -0.026710000000000001 -0.024910000000000002 -0.024199999999999999 -0.023570000000000001 -0.023449999999999999]  InternalRulePriority=Speed  RndMeth=Simplest
      settings: InputPortMap=u0,u1
  Cm_q1 : Lookup_n-D  BreakpointsForDimension1=[-4;4;12;20]  BreakpointsForDimension2=[0.4;3.2]  BreakpointsForDimension3=[0;10;20;30]  Table=[-0.3076582 -0.2329223;-0.3207673 -0.2427394;-0.3456418 -0.2478269;-0.3821332 -0.2480956]  InternalRulePriority=Speed  RndMeth=Simplest
      settings: InputPortMap=u0,u1
  Cmtable : Lookup_n-D  BreakpointsForDimension1=[-10;-5;0;5;10;15;20]  BreakpointsForDimension2=[0;0.40000000000000002;0.59999999999999998;0.80000000000000004;0.90000000000000002;0.94999999999999996;1;1.05;1.1000000000000001;1.1499999999999999;1.2;1.3999999999999999;1.6000000000000001;1.8;2;2.2000000000000002;2.3999999999999999;2.6000000000000001;2.7999999999999998;3;3.2000000000000002;3.3999999999999999;3.6000000000000001;3.7999999999999998;4]  BreakpointsForDimension3=[0;10;20;30]  Table=[0.032176000000000003 0.032176000000000003 0.039531999999999998 0.047910000000000001 0.055923 0.055632000000000001 0.074579999999999994 0.075497999999999996 0.073704000000000006 0.072221999999999995 0.069863999999999996 0.059761000000000002 0.050795 0.044049999999999999 0.038963999999999999 0.034888000000000002 0.031623999999999999 0.028850000000000001 0.026443000000000001 0.024421999999999999 0.022709 0.022709 0.022709 0.022709 0.022709;0.012319999999999999 0.012319999999999999 0.012925000000000001 0.014788000000000001 0.017801000000000001 0.023310999999999998 0.035723999999999999 0.039172999999999999 0.038981000000000002 0.038662000000000002 0.038066999999999997 0.034171 0.029125000000000002 0.024944999999999998 0.021666000000000001 0.019282000000000001 0.017461000000000001 0.015966999999999999 0.014687 0.013608 0.012694 0.011849999999999999 0.011096 0.010297000000000001 0.0098549999999999992;-0.00197 -0.00197 -0.0027200000000000002 -0.0046800000000000001 -0.0078200000000000006 -0.0020699999999999998 0.0090119999999999992 0.010406 0.011159000000000001 0.011518 0.011563 0.010671 0.0088800000000000007 0.0071510000000000002 0.005659 0.0045409999999999999 0.003728 0.0032169999999999998 0.0029399999999999999 0.0027950000000000002 0.0027049999999999999 0.0026540000000000001 0.0026540000000000001 0.002562 0.002529;-0.017809999999999999 -0.017809999999999999 -0.019640000000000001 -0.023120000000000002 -0.029790000000000001 -0.032439999999999997 -0.01443 -0.01694 -0.014789999999999999 -0.012749999999999999 -0.01238 -0.01073 -0.01064 -0.010279999999999999 -0.0099399999999999992 -0.0095300000000000003 -0.0089999999999999993 -0.00843 -0.0078200000000000006 -0.0071999999999999998 -0.0064700000000000001 -0.0058700000000000002 -0.00528 -0.0047699999999999999 -0.0042700000000000004;-0.029499999999999998 -0.029499999999999998 -0.036069999999999998 -0.04258 -0.050299999999999997 -0.054579999999999997 -0.042419999999999999 -0.043470000000000002 -0.042009999999999999 -0.040050000000000002 -0.037089999999999998 -0.032739999999999998 -0.030169999999999999 -0.02784 -0.025350000000000001 -0.023 -0.02094 -0.019109999999999999 -0.017489999999999999 -0.016060000000000001 -0.01472 -0.01355 -0.01252 -0.011560000000000001 -0.01043;-0.044200000000000003 -0.044200000000000003 -0.052299999999999999 -0.055579999999999997 -0.065820000000000004 -0.075420000000000001 -0.078700000000000006 -0.075190000000000007 -0.070949999999999999 -0.068360000000000004 -0.064850000000000005 -0.054620000000000002 -0.048309999999999999 -0.043650000000000001 -0.039469999999999998 -0.035630000000000002 -0.032370000000000003 -0.02937 -0.026880000000000001 -0.024910000000000002 -0.023120000000000002 -0.021680000000000001 -0.021680000000000001 -0.01899 -0.01787;-0.061609999999999998 -0.061609999999999998 -0.062170000000000003 -0.072059999999999999 -0.090200000000000002 -0.09801 -0.10750999999999999 -0.10460999999999999 -0.10123 -0.096879999999999994 -0.091619999999999993 -0.077240000000000003 -0.067080000000000001 -0.059749999999999998 -0.053670000000000002 -0.048750000000000002 -0.044769999999999997 -0.040890000000000003 -0.037620000000000001 -0.034869999999999998 -0.032530000000000003 -0.032530000000000003 -0.029090000000000001 -0.027640000000000001 -0.026360000000000001]  InternalRulePriority=Speed  RndMeth=Simplest
      settings: InputPortMap=u0,u1
  Divide : Product  Inputs=*/
  Divide1 : Product  Inputs=*/
  Gain10 : Gain  Gain=2
  Gain11 : Gain  Gain=c
  Gain12 : Gain  Gain=2
  Gain2 : Gain  Gain=Cm_AlphaDot
  Gain9 : Gain  Gain=c
  Product1 : Product
  Product2 : Product
  Scope : Scope
      settings: ActiveDisplayYMinimum=-0.00093867796621814256  ActiveDisplayYMaximum=0.039401193688923558
  Scope5 : Scope
      settings: ActiveDisplayYMinimum=-0.03679  ActiveDisplayYMaximum=0.03001  DataLoggingVariableName=ScopeData8
  Cms : Outport
  wires:
  Angle Conversion3/1 -> Cm_q1/1
  mach/1 -> Cm_q1/2, Gain10/1, Gain12/1, Cm_elev/2, Cmtable/2
  Elevator_rad/1 -> Product1/2
  Angle Conversion1/1 -> Cmtable/1
  Cm_elev/1 -> Product1/1
  AlphaDot_radps/1 -> Gain2/1
  Divide1/1 -> ?
  Alpha_rad/1 -> Angle Conversion1/1, Angle Conversion3/1, Angle Conversion2/1
  Angle Conversion2/1 -> Cm_elev/1
  Gain2/1 -> Gain11/1
  q_radps/1 -> Product2/1
  Gain11/1 -> Divide1/1
  Cm_q1/1 -> Product2/2
  Gain12/1 -> Divide1/2
  Cmtable/1 -> Add/1
  Product1/1 -> Add/2, Scope5/1
  Product2/1 -> Gain9/1
  Gain9/1 -> Divide/1
  Gain10/1 -> Divide/2
  Divide/1 -> ?
  Add/1 -> Cms/1, Scope/1
